simulink model "gmp_pmsm_sil_mdl"  (R2024b)
settings: Solver=VariableStepAuto  StartTime=0.0  StopTime=2  RelTol=1e-3
libraries: peripheral_utilities x11, spsSeriesRLCBranchLib x6, spsControlledVoltageSourceLib x1, gmp_sil_core_pack x1, spsGroundLib x1, spsPermanentMagnetSynchronousMachineLib x1, sps_lib x1, spspowerguiLib x1
settings Model: Creator=javnson  LastModifiedBy=javnson
settings OptimizationCC: ReuseModelBlockBuffer=off
settings RTWCC: GPUComputeCapability=3.5

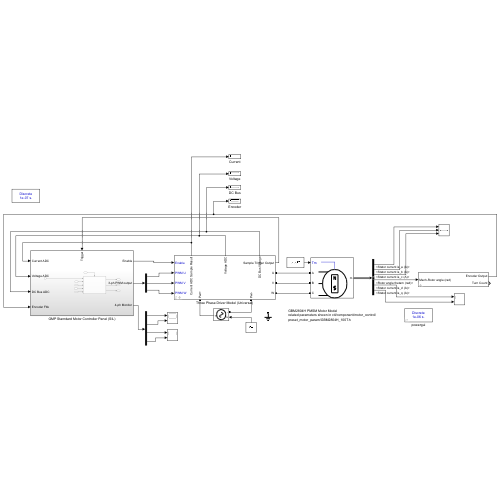
[thumbnail: Simulink's stored preview of the top-level diagram]
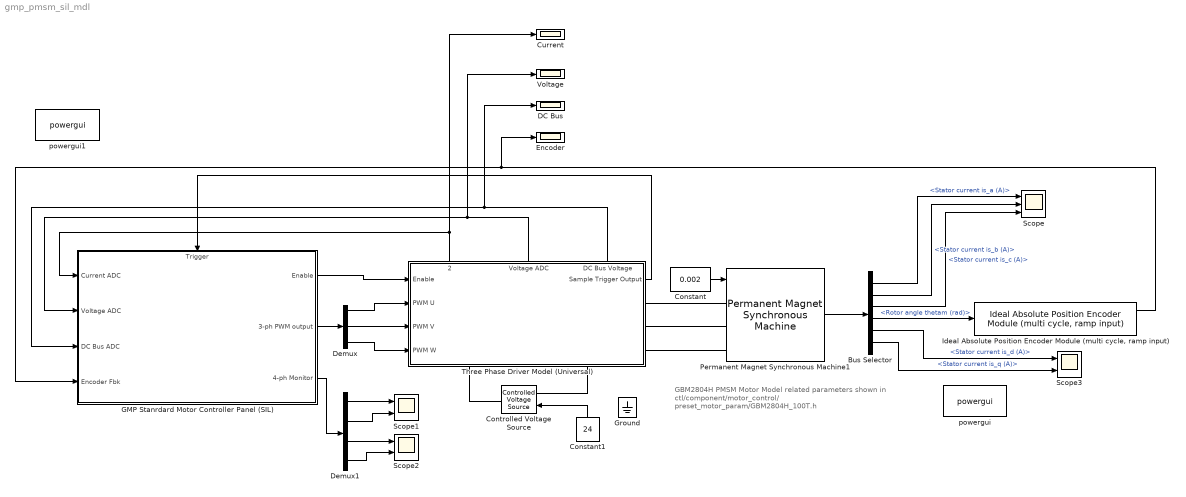
== system gmp_pmsm_sil_mdl ==
  note: GBM2804H PMSM Motor Model
      | related parameters shown in ctl/component/motor_control/
      | preset_motor_param/GBM2804H_100T.h
  Bus Selector : BusSelector  OutputSignals=Stator current is_a (A),Stator current is_b (A),Stator current is_c (A),Rotor angle thetam (rad),Stator current is_d (A),Stator current is_q (A)
  Constant : Constant  Value=0.002
  Constant1 : Constant  Value=24
  Controlled Voltage Source : spsControlledVoltageSourceLib/Controlled Voltage Source  Initialize=on  Source_Type=AC  Amplitude=0  Phase=0  Frequency=0  Measurements=None
  Current : Scope
  DC Bus : Scope
  Demux : Demux  Outputs=3
  Demux1 : Demux
  Encoder : Scope
  GMP Stanrdard Motor Controller Panel (SIL) : Subsystem
      settings: PortSchema="{\"entries\":[{\"content\":{\"sides\":[{\"content\":{\"connectorIds\":[\"In1\",\"In2\",\"In3\",\"In4\"]},\"type\":\"ConnectorPlacement.EquallySpacedRectSide\",\"uuid\":\"92070e77-c4d8-4bd6-a20f-015d90d53703\"},{\"content\":{\"connectorIds\":[\"Out1\",\"Out2\",\"Out3\"],\"side\":\"RIGHT\"},\"type\":\"ConnectorPlacement.EquallySpacedRectSide\",\"uuid\":\"cd227558-01ea-4976-b12d-cc815f5c8239\"},{\"content\":{\"connectorIds\":[\"In5\"],\"side\":\"TOP\"},\"type\":\"ConnectorPlacement.EquallySpacedRectSide\",\"uuid\":\"6d86fdab-8964-4d81-bb99-d1a603f01c68\"}]},\"type\":\"ConnectorPlacement.EquallySpacedConnector\",\"uuid\":\"4dd76185-b108-46e1-8d6d-0c6e9edd0ad4\"}],\"packageUris\":[\"http://schema.mathworks.com/mf0/Connector/R2020b\"],\"version\":\"1.0\"}"
  Ground : spsGroundLib/Ground  LConnTagsString=a
  "Ideal Absolute Position Encoder Module (multi cycle, ramp input)" : peripheral_utilities/Ideal Absolute Position Encoder Module (multi cycle, ramp input)  ENCODER_BIT=14
      settings: SourceProductName=Virtual Peripheral Utilities
  Permanent Magnet Synchronous Machine1 : spsPermanentMagnetSynchronousMachineLib/Permanent Magnet Synchronous Machine  NbPhases=3  FluxDistribution=Sinusoidal  RotorType=Round  MechanicalLoad=Torque Tm  PresetModel=No  ShowDetailedParameters=on  MeasurementBus=off  Resistance=4.7  Inductance=8.5e-3  dqInductances=[8.5e-3,8.5e-3]  La=0.96e-3  MachineConstant=Voltage Constant (V_peak L-L / krpm)  Flux=0.0038197  VoltageCst=1000/206.2  TorqueCst=0.040106  Flat=120  Mechanical=[497e-9 755e-9 7 0]  PolePairs=4  InitialConditions=[0, 0, 0, 0]  InitialConditions5ph=[0 0 0 0 0 0]  RefAngle=Aligned with phase A axis (original Park)  IterativeDiscreteModel=Trapezoidal non iterative  TsBlock=-1  TsPowergui=0
  Scope : Scope  NumInputPorts=3
  Scope1 : Scope  NumInputPorts=2
  Scope2 : Scope  NumInputPorts=2
  Scope3 : Scope  NumInputPorts=2
  Three Phase Driver Model (Universal) : Subsystem  AncestorBlock=peripheral_utilities/Three Phase Driver Model (Universal)  mask{fswitch=10e3, CMP_MAX=6000, Deadband_Upper=75, Deadband_Lower=75, Deadband_us=1.25, phase_shift=0, R_mosfet_on=0.1, Lon=0, Rd=0.01, Vf=0.3, Rs=1e5, Cs=inf, Rsap=0.005, ADC_GAIN=20, ADC_BIT=12, ADC_REFERENCE=3.3, ADC_BIAS=1.65, ADC_INIT=0, VOLTAGE_ADC_GAIN=0.04049127, VOLTAGE_ADC_BIT=12, VOLTAGE_ADC_REFERENCE=3.3, VOLTAGE_ADC_VOLTAGE=0, VOLTAGE_ADC_INIT=0, VOLTAGE_ADC_CUT_FREQ=1143.4, DCBUS_ADC_GAIN=0.04049127, DCBUS_ADC_BIT=12, DCBUS_ADC_REFERENCE=3.3, DCBUS_ADC_BIAS=0, DCBUS_ADC_INIT=0}
      mask init:
      | calculate_deadband(gcb, 'Deadband_Upper', 'Deadband_Lower',	'CMP_MAX', 'fswitch', 'Deadband_us');
      settings: PortSchema="{\"entries\":[{\"content\":{\"sides\":[{\"content\":{\"connectorIds\":[\"In1\",\"In2\",\"In3\",\"In4\"]},\"type\":\"ConnectorPlacement.EquallySpacedRectSide\",\"uuid\":\"3f4c86ad-0582-4f47-8583-a8af9a7f9adc\"},{\"content\":{\"connectorIds\":[\"Out1\",\"RConn1\",\"RConn2\",\"RConn3\"],\"side\":\"RIGHT\"},\"type\":\"ConnectorPlacement.EquallySpacedRectSide\",\"uuid\":\"ae91f325-3014-4188-9063-296f4d5623fa\"},{\"content\":{\"connectorIds\":[\"Out2\",\"Out3\",\"Out4\"],\"side\":\"TOP\"},\"type\":\"ConnectorPlacement.EquallySpacedRectSide\",\"uuid\":\"5f2edb36-6849-4a72-b7bd-4d267f120ce4\"},{\"content\":{\"connectorIds\":[\"RConn4\",\"RConn5\"],\"side\":\"BOTTOM\"},\"type\":\"ConnectorPlacement.EquallySpacedRectSide\",\"uuid\":\"79a111ed-6591-4ced-9242-67ea1247c580\"}]},\"type\":\"ConnectorPlacement.EquallySpacedConnector\",\"uuid\":\"8c66eb8e-d25c-472f-a4a5-d1759225ba1c\"}],\"packageUris\":[\"http://schema.mathworks.com/mf0/Connector/R2020b\"],\"version\":\"1.0\"}"
      mask Callback fswitch: calculate_deadband(gcb, 'Deadband_Upper', 'Deadband_Lower',	'CMP_MAX', 'fswitch', 'Deadband_us');
      mask Callback CMP_MAX: calculate_deadband(gcb, 'Deadband_Upper', 'Deadband_Lower',	'CMP_MAX', 'fswitch', 'Deadband_us');
      mask Callback Deadband_Upper: calculate_deadband(gcb, 'Deadband_Upper', 'Deadband_Lower',	'CMP_MAX', 'fswitch', 'Deadband_us');
      mask Callback Deadband_Lower: calculate_deadband(gcb, 'Deadband_Upper', 'Deadband_Lower',	'CMP_MAX', 'fswitch', 'Deadband_us');
      mask DialogControl DescGroupVar Prompt: Three Phases Bridge Peripheral(3-shunt sample)
      mask DialogControl Control21 Prompt: GMP CTL Simulink Utilities: virtual peripherals
      mask DialogControl DescTextVar Prompt: This module provide a ideal 3-phases bridge peripheral.
      mask DialogControl Container4 Prompt: PWM config
      mask DialogControl ParameterGroupVar Prompt: PWM parameters
      mask DialogControl Control2 Prompt: PWM Frequency (Hz):
      mask DialogControl Control4 Prompt: Full Scale PWM Compare value:
      mask DialogControl Control5 Prompt: Deadband Range Set (CMP Value):
      mask DialogControl Control6 Prompt: Deadband time: DEADBAND_CMP/2/CMP_MAX/fswitch
      mask DialogControl Control22 Prompt: Calculated Deadband, us
      mask DialogControl Control20 Prompt: Initial Phase shift:
      mask DialogControl Container5 Prompt: MOSFET config
      mask DialogControl Container7 Prompt: MOSFET parameters
      mask DialogControl Control7 Prompt: Rds(on), unit Ohm
      mask DialogControl Control8 Prompt: Internal diode inducctance, unit H
      mask DialogControl Control9 Prompt: Internal diode resistance Rd, unit Ohm
      mask DialogControl Control10 Prompt: Internal diode forward voltage Vf, unit V
      mask DialogControl Control11 Prompt: Snubber resistance Rs, unit ohm
      mask DialogControl Control12 Prompt: Snubber Capacitance Cs, unit F
      mask DialogControl Container6 Prompt: 3-shunt Current Sample
      mask DialogControl Control13 Prompt: ADC(p.u.) = (real_voltage * ADC_GAIN + ADC_BIAS)/ADC_REFERENCE
      mask DialogControl Control15 Prompt: Shunt Smaple Res, unit Ohm
      mask DialogControl Control14 Prompt: ADC Voltage Gain (Scale Factor):
      mask DialogControl Control16 Prompt: ADC resolution:
      mask DialogControl Control17 Prompt: ADC reference Voltage(V)
      mask DialogControl Control18 Prompt: ADC Bias Voltage(V)
      mask DialogControl Control19 Prompt: ADC Initial Voltage Output (V):
      mask DialogControl Container9 Prompt: 3-shunt Voltage Sample
      mask DialogControl Control34 Prompt: ADC Voltage Gain (Scale Factor):
      mask DialogControl Control23 Prompt: ADC resolution:
      mask DialogControl Control24 Prompt: ADC reference voltage (V), when VOLTAGE_ADC_GAIN = 1, ADC_REF = ADC Full scale
      mask DialogControl Control25 Prompt: ADC Bias Voltage (V):
      mask DialogControl Control26 Prompt: ADC Initial Voltage Output (V):
      mask DialogControl Control27 Prompt: Voltage Filter cut frequency (Hz):
      mask DialogControl Control28 Prompt: Generally, this value less than switch frequency / 10, greater than motor normal frequency * 3
      mask DialogControl Container10 Prompt: DC Bus Voltage Sample
      mask DialogControl Control32 Prompt: ADC reference voltage (V), when VOLTAGE_ADC_GAIN = 1, ADC_REF = ADC Full scale
      mask DialogControl Control29 Prompt: ADC Voltage Gain (Scale Factor):
      mask DialogControl Control30 Prompt: ADC resolution:
      mask DialogControl Control31 Prompt: ADC Bias Voltage (V):
      mask DialogControl Control33 Prompt: ADC Initial Voltage Output (V):
  Voltage : Scope
  powergui : sps_lib/powergui  Priority=1  SimulationMode=Discrete  SampleTime=1e-6  frequency=60  Iterations=50  frequencyindice=0  Pbase=100e6  ErrMax=1e-4  UnitsV=kV  UnitsW=MW  buscounter=0  FunctionMessages=off  echomessages=off  EnableUseOfTLC=off  CurrentSourceSwitches=off  DisableSnubberDevices=off  DisableRonSwitches=off  DisableVfSwitches=off  DisplayEquations=off  AutomaticDiscreteSolvers=off  SolverType=Tustin/Backward Euler (TBE)  Interpol=off  ExternalGateDelay=off  methode=off  Ts=100  x0status=blocks  SPID=on  SwTol=0  HookPort=off  NonlinearTolerance=1e-4  nMaxIteration=100  ContinueOnMaxIteration=off  RestoreLinks=warning  ResistiveCurrentMeasurement=off  Frange=[0:2:500]  Ylog=off  Xlog=on  ShowGrid=off  save=off  variable=ZData  structure=0  ZoomFFT=off  StartTime=0.0  cycles=1  DisplayStyle=1  fundamental=60  FreqAxis=off  MaxFrequency=1000  frequencyindicesteady=1  RmsSteady=1  display=off
  powergui1 : spspowerguiLib/powergui  Priority=1  SimulationMode=Discrete  SampleTime=1e-7  frequency=60  Iterations=50  frequencyindice=60  Pbase=100e6  ErrMax=1e-4  UnitsV=kV  UnitsW=MW  buscounter=0  FunctionMessages=off  echomessages=off  EnableUseOfTLC=off  CurrentSourceSwitches=off  DisableSnubberDevices=off  DisableRonSwitches=off  DisableVfSwitches=off  DisplayEquations=off  AutomaticDiscreteSolvers=off  SolverType=Tustin/Backward Euler (TBE)  Interpol=off  ExternalGateDelay=off  methode=off  Ts=100  x0status=blocks  SPID=on  SwTol=0  HookPort=off  NonlinearTolerance=1e-4  nMaxIteration=100  ContinueOnMaxIteration=off  RestoreLinks=warning  ResistiveCurrentMeasurement=off  Frange=[0:2:500]  Ylog=off  Xlog=on  ShowGrid=off  save=off  variable=ZData  structure=0  ZoomFFT=off  StartTime=0.0  cycles=1  DisplayStyle=1  fundamental=60  FreqAxis=off  MaxFrequency=1000  frequencyindicesteady=1  RmsSteady=1  display=off
  wires:
  Constant/1 -> Permanent Magnet Synchronous Machine1/1
  Bus Selector/1 -> Scope/1  "<Stator current is_a (A)>"
  Bus Selector/2 -> Scope/2  "<Stator current is_b (A)>"
  Bus Selector/3 -> Scope/3  "<Stator current is_c (A)>"
  Demux/1 -> Three Phase Driver Model (Universal)/2(PWM U)
  Demux/2 -> Three Phase Driver Model (Universal)/3(PWM V)
  Demux/3 -> Three Phase Driver Model (Universal)/4(PWM W)
  Constant1/1 -> Controlled Voltage Source/1
  Bus Selector/4 -> "Ideal Absolute Position Encoder Module (multi cycle, ramp input)"/1  "<Rotor angle thetam (rad)>"
  Three Phase Driver Model (Universal)/2(Current ADC Sample Result) -> Current/1, GMP Stanrdard Motor Controller Panel (SIL)/1(Current ADC)
  Three Phase Driver Model (Universal)/3(Voltage ADC) -> Voltage/1, GMP Stanrdard Motor Controller Panel (SIL)/2(Voltage ADC)
  "Ideal Absolute Position Encoder Module (multi cycle, ramp input)"/1 -> GMP Stanrdard Motor Controller Panel (SIL)/4(Encoder Fbk), Encoder/1
  GMP Stanrdard Motor Controller Panel (SIL)/1(Enable) -> Three Phase Driver Model (Universal)/1(Enable)
  GMP Stanrdard Motor Controller Panel (SIL)/2(3-ph PWM output) -> Demux/1
  GMP Stanrdard Motor Controller Panel (SIL)/3(4-ph Monitor) -> Demux1/1
  Three Phase Driver Model (Universal)/1(Sample Trigger Output) -> GMP Stanrdard Motor Controller Panel (SIL)/5(Trigger)
  Three Phase Driver Model (Universal)/4(DC Bus Voltage) -> GMP Stanrdard Motor Controller Panel (SIL)/3(DC Bus ADC), DC Bus/1
  Permanent Magnet Synchronous Machine1/1 -> Bus Selector/1
  Demux1/1 -> Scope1/1
  Demux1/2 -> Scope1/2
  Demux1/3 -> Scope2/1
  Demux1/4 -> Scope2/2
  Bus Selector/5 -> Scope3/1  "<Stator current is_d (A)>"
  Bus Selector/6 -> Scope3/2  "<Stator current is_q (A)>"
  connections:
  Permanent Magnet Synchronous Machine1/LConn1 -- Three Phase Driver Model (Universal)/RConn1
  Permanent Magnet Synchronous Machine1/LConn2 -- Three Phase Driver Model (Universal)/RConn2
  Permanent Magnet Synchronous Machine1/LConn3 -- Three Phase Driver Model (Universal)/RConn3
  Three Phase Driver Model (Universal)/RConn4 -- Controlled Voltage Source/RConn1
  Three Phase Driver Model (Universal)/RConn5 -- Controlled Voltage Source/LConn1

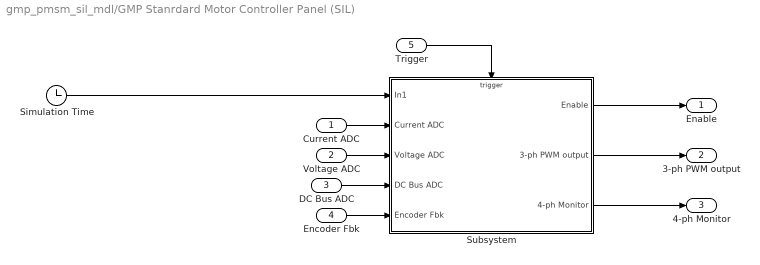
== system gmp_pmsm_sil_mdl/GMP Stanrdard Motor Controller Panel (SIL) ==
  Current ADC : Inport
  Voltage ADC : Inport  Port=2
  DC Bus ADC : Inport  Port=3
  Encoder Fbk : Inport  Port=4
  Trigger : Inport  Port=5
  Simulation Time : Clock
  Subsystem : Subsystem
  Enable : Outport
  3-ph PWM output : Outport  Port=2
  4-ph Monitor : Outport  Port=3
  wires:
  Simulation Time/1 -> Subsystem/1(In1)
  Current ADC/1 -> Subsystem/2(Current ADC)
  Voltage ADC/1 -> Subsystem/3(Voltage ADC)
  DC Bus ADC/1 -> Subsystem/4(DC Bus ADC)
  Encoder Fbk/1 -> Subsystem/5(Encoder Fbk)
  Subsystem/1(Enable) -> Enable/1
  Subsystem/2(3-ph PWM output) -> 3-ph PWM output/1
  Subsystem/3(4-ph Monitor) -> 4-ph Monitor/1
  Trigger/1 -> Subsystem/Trigger

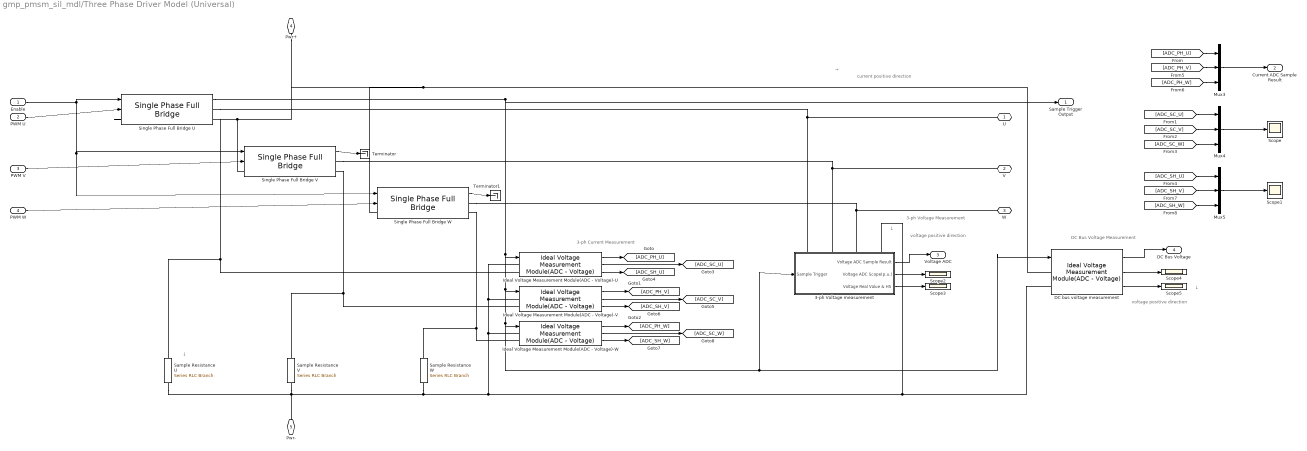
== system gmp_pmsm_sil_mdl/Three Phase Driver Model (Universal) ==
  note: voltage positive direction
  note: ↓
  note: DC Bus Voltage Measurement
  note: 3-ph Voltage Measurement
  note: ↓
  note: voltage positive direction
  note: ↓
  note: current positive direction
  note: →
  note: 3-ph Current Measurement
  Enable : Inport
  PWM U : Inport  Port=2
  PWM V : Inport  Port=3
  PWM W : Inport  Port=4
  3-ph Voltage measurement : Subsystem  AncestorBlock=peripheral_utilities/Three Phases Voltage (ph-gnd) Measurement with Filter  mask{ADC_GAIN=VOLTAGE_ADC_GAIN, ADC_BIT=VOLTAGE_ADC_BIT, ADC_REFERENCE=VOLTAGE_ADC_REFERENCE, ADC_BIAS=VOLTAGE_ADC_VOLTAGE, ADC_INIT=VOLTAGE_ADC_INIT, cut_frequency=VOLTAGE_ADC_CUT_FREQ}
      settings: PortSchema="{\"entries\":[{\"content\":{\"sides\":[{\"content\":{\"connectorIds\":[\"In1\"]},\"type\":\"ConnectorPlacement.EquallySpacedRectSide\",\"uuid\":\"ae4f4612-c092-4fa0-8a43-5c9e823110e3\"},{\"content\":{\"connectorIds\":[\"Out1\",\"Out2\",\"Out3\"],\"side\":\"RIGHT\"},\"type\":\"ConnectorPlacement.EquallySpacedRectSide\",\"uuid\":\"6db15ef0-d33a-4775-b4e6-14a566796673\"},{\"content\":{\"connectorIds\":[\"LConn1\",\"LConn2\",\"LConn3\",\"LConn4\"],\"side\":\"TOP\"},\"type\":\"ConnectorPlacement.EquallySpacedRectSide\",\"uuid\":\"cfddd664-59f3-497b-b33e-fe832fe7a7bd\"}]},\"type\":\"ConnectorPlacement.EquallySpacedConnector\",\"uuid\":\"5bacf0ad-0c4a-4f47-a242-d8a476ab7f52\"}],\"packageUris\":[\"http://schema.mathworks.com/mf0/Connector/R2020b\"],\"version\":\"1.0\"}"
      mask DialogControl DescGroupVar Prompt: 3 phases Voltage Sample ADC Model
      mask DialogControl Control10 Prompt: GMP CTL Simulink Utilities: virtual peripherals
      mask DialogControl DescTextVar Prompt: This is a ideal Voltage Measurement Module.
      mask DialogControl Control2 Prompt: ADC(p.u.) = (real_voltage * ADC_GAIN + ADC_BIAS)/ADC_REFERENCE
      mask DialogControl ParameterGroupVar Prompt: parameters:
      mask DialogControl Control3 Prompt: ADC Voltage Gain (Scale Factor):
      mask DialogControl Control4 Prompt: ADC resolution:
      mask DialogControl Control5 Prompt: ADC reference Voltage (V), when ADC_GAIN=1, ADC_REF = ADC full scale
      mask DialogControl Control6 Prompt: ADC Bias Voltage(V)
      mask DialogControl Control7 Prompt: ADC Initial Voltage Output (V):
      mask DialogControl Control8 Prompt: Voltage Filter cut frequency (Hz):
      mask DialogControl Control9 Prompt: Generally, this value less than switch frequency / 10, greater than motor normal frequency * 3
  DC bus voltage measurement : peripheral_utilities/Ideal Voltage Measurement Module(ADC - Voltage)  ADC_GAIN=DCBUS_ADC_GAIN  ADC_BIT=DCBUS_ADC_BIT  ADC_REFERENCE=DCBUS_ADC_REFERENCE  ADC_BIAS=DCBUS_ADC_BIAS  ADC_INIT=DCBUS_ADC_INIT
      settings: SourceProductName=Virtual Peripheral Utilities
  Ideal Voltage Measurement Module(ADC - Voltage)-U : peripheral_utilities/Ideal Voltage Measurement Module(ADC - Voltage)  ADC_GAIN=ADC_GAIN  ADC_BIT=ADC_BIT  ADC_REFERENCE=ADC_REFERENCE  ADC_BIAS=ADC_BIAS  ADC_INIT=ADC_INIT
      settings: SourceProductName=Virtual Peripheral Utilities
  Ideal Voltage Measurement Module(ADC - Voltage)-V : peripheral_utilities/Ideal Voltage Measurement Module(ADC - Voltage)  ADC_GAIN=ADC_GAIN  ADC_BIT=ADC_BIT  ADC_REFERENCE=ADC_REFERENCE  ADC_BIAS=ADC_BIAS  ADC_INIT=ADC_INIT
      settings: SourceProductName=Virtual Peripheral Utilities
  Ideal Voltage Measurement Module(ADC - Voltage)-W : peripheral_utilities/Ideal Voltage Measurement Module(ADC - Voltage)  ADC_GAIN=ADC_GAIN  ADC_BIT=ADC_BIT  ADC_REFERENCE=ADC_REFERENCE  ADC_BIAS=ADC_BIAS  ADC_INIT=ADC_INIT
      settings: SourceProductName=Virtual Peripheral Utilities
  Mux3 : Mux  Inputs=3
  Mux4 : Mux  Inputs=3
  Mux5 : Mux  Inputs=3
  Sample Resistance U : spsSeriesRLCBranchLib/Series RLC Branch  LConnTagsString=__new0  RConnTagsString=__new0  BranchType=R  Resistance=Rsap  Inductance=1e-3  SetiL0=off  InitialCurrent=0  Capacitance=1e-6  Setx0=off  InitialVoltage=0  Measurements=None
  Sample Resistance V : spsSeriesRLCBranchLib/Series RLC Branch  LConnTagsString=__new0  RConnTagsString=__new0  BranchType=R  Resistance=Rsap  Inductance=1e-3  SetiL0=off  InitialCurrent=0  Capacitance=1e-6  Setx0=off  InitialVoltage=0  Measurements=None
  Sample Resistance W : spsSeriesRLCBranchLib/Series RLC Branch  LConnTagsString=__new0  RConnTagsString=__new0  BranchType=R  Resistance=Rsap  Inductance=1e-3  SetiL0=off  InitialCurrent=0  Capacitance=1e-6  Setx0=off  InitialVoltage=0  Measurements=None
  Scope{,1..5} (6 alike) : Scope
  Single Phase Full Bridge U : peripheral_utilities/Single Phase Full Bridge  fswitch=fswitch  CMP_MAX=CMP_MAX  Deadband_Upper=Deadband_Upper  Deadband_Lower=Deadband_Lower  Deadband_us=NaN  phase_shift=phase_shift  R_mosfet_on=R_mosfet_on  Lon=Lon  Rd=Rd  Vf=Vf  Rs=Rs  Cs=Cs
      settings: SourceProductName=Virtual Peripheral Utilities
  Single Phase Full Bridge V : peripheral_utilities/Single Phase Full Bridge  fswitch=fswitch  CMP_MAX=CMP_MAX  Deadband_Upper=Deadband_Upper  Deadband_Lower=Deadband_Lower  Deadband_us=NaN  phase_shift=phase_shift  R_mosfet_on=R_mosfet_on  Lon=Lon  Rd=Rd  Vf=Vf  Rs=Rs  Cs=Cs
      settings: SourceProductName=Virtual Peripheral Utilities
  Single Phase Full Bridge W : peripheral_utilities/Single Phase Full Bridge  fswitch=fswitch  CMP_MAX=CMP_MAX  Deadband_Upper=Deadband_Upper  Deadband_Lower=Deadband_Lower  Deadband_us=NaN  phase_shift=phase_shift  R_mosfet_on=R_mosfet_on  Lon=Lon  Rd=Rd  Vf=Vf  Rs=Rs  Cs=Cs
      settings: SourceProductName=Virtual Peripheral Utilities
  Terminator : Terminator
  Terminator1 : Terminator
  U : PMIOPort  Side=Right
  V : PMIOPort  Port=2  Side=Right
  W : PMIOPort  Port=3  Side=Right
  Pwr+ : PMIOPort  Port=4  Side=Right
  Pwr- : PMIOPort  Port=5  Side=Right
  Sample Trigger Output : Outport
  Current ADC Sample Result : Outport  Port=2
  Voltage ADC : Outport  Port=3
  DC Bus Voltage : Outport  Port=4
  wires:
  DC bus voltage measurement/3 -> Scope5/1
  DC bus voltage measurement/2 -> Scope4/1
  DC bus voltage measurement/1 -> DC Bus Voltage/1
  3-ph Voltage measurement/3(Voltage Real Value & HS) -> Scope3/1
  3-ph Voltage measurement/2(Voltage ADC Scope(p.u.)) -> Scope2/1
  3-ph Voltage measurement/1(Voltage ADC Sample Result) -> Voltage ADC/1
  Ideal Voltage Measurement Module(ADC - Voltage)-W/2 -> [ADC_SC_W]
  [ADC_SH_V] -> Mux5/2
  [ADC_SC_W] -> Mux4/3
  [ADC_PH_W] -> Mux3/3
  Ideal Voltage Measurement Module(ADC - Voltage)-W/3 -> [ADC_SH_W]
  Ideal Voltage Measurement Module(ADC - Voltage)-V/2 -> [ADC_SC_V]
  [ADC_SH_U] -> Mux5/1
  Single Phase Full Bridge U/1 -> Sample Trigger Output/1, Ideal Voltage Measurement Module(ADC - Voltage)-U/1, 3-ph Voltage measurement/1(Sample Trigger), DC bus voltage measurement/1, Ideal Voltage Measurement Module(ADC - Voltage)-W/1, Ideal Voltage Measurement Module(ADC - Voltage)-V/1
  Ideal Voltage Measurement Module(ADC - Voltage)-V/3 -> [ADC_SH_V]
  Mux4/1 -> Scope/1
  Enable/1 -> Single Phase Full Bridge U/1, Single Phase Full Bridge W/1, Single Phase Full Bridge V/1
  [ADC_PH_U] -> Mux3/1
  Ideal Voltage Measurement Module(ADC - Voltage)-W/1 -> [ADC_PH_W]
  Mux5/1 -> Scope1/1
  [ADC_SH_W] -> Mux5/3
  [ADC_SC_U] -> Mux4/1
  Ideal Voltage Measurement Module(ADC - Voltage)-V/1 -> [ADC_PH_V]
  Mux3/1 -> Current ADC Sample Result/1
  Ideal Voltage Measurement Module(ADC - Voltage)-U/3 -> [ADC_SH_U]
  [ADC_SC_V] -> Mux4/2
  [ADC_PH_V] -> Mux3/2
  PWM W/1 -> Single Phase Full Bridge W/2
  PWM V/1 -> Single Phase Full Bridge V/2
  Ideal Voltage Measurement Module(ADC - Voltage)-U/2 -> [ADC_SC_U]
  Single Phase Full Bridge W/1 -> Terminator1/1
  Single Phase Full Bridge V/1 -> Terminator/1
  Ideal Voltage Measurement Module(ADC - Voltage)-U/1 -> [ADC_PH_U]
  PWM U/1 -> Single Phase Full Bridge U/2
  connections:
  Single Phase Full Bridge V/LConn1 -- Single Phase Full Bridge U/LConn1 -- DC bus voltage measurement/LConn1 -- Single Phase Full Bridge W/LConn1 -- Pwr+/RConn1
  Single Phase Full Bridge U/RConn2 -- Ideal Voltage Measurement Module(ADC - Voltage)-U/LConn2 -- Sample Resistance U/LConn1
  Single Phase Full Bridge W/RConn2 -- Ideal Voltage Measurement Module(ADC - Voltage)-W/LConn2 -- Sample Resistance W/LConn1
  Ideal Voltage Measurement Module(ADC - Voltage)-W/LConn1 -- Ideal Voltage Measurement Module(ADC - Voltage)-V/LConn1 -- Ideal Voltage Measurement Module(ADC - Voltage)-U/LConn1 -- DC bus voltage measurement/LConn2 -- 3-ph Voltage measurement/LConn4 -- Sample Resistance W/RConn1 -- Sample Resistance V/RConn1 -- Sample Resistance U/RConn1 -- Pwr-/RConn1
  Single Phase Full Bridge V/RConn2 -- Ideal Voltage Measurement Module(ADC - Voltage)-V/LConn2 -- Sample Resistance V/LConn1
  3-ph Voltage measurement/LConn3 -- W/RConn1 -- Single Phase Full Bridge W/RConn1
  3-ph Voltage measurement/LConn1 -- U/RConn1 -- Single Phase Full Bridge U/RConn1
  3-ph Voltage measurement/LConn2 -- V/RConn1 -- Single Phase Full Bridge V/RConn1

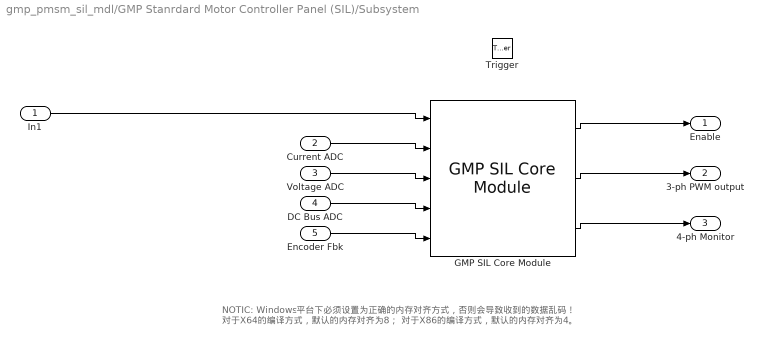
== system gmp_pmsm_sil_mdl/GMP Stanrdard Motor Controller Panel (SIL)/Subsystem ==
  note: NOTIC:
      | Windows平台下必须设置为正确的内存对齐方式，否则会导致收到的数据乱码！
      | 对于X64的编译方式，默认的内存对齐为8；
      | 对于X86的编译方式，默认的内存对齐为4。
  In1 : Inport
  Current ADC : Inport  Port=2
  Voltage ADC : Inport  Port=3
  DC Bus ADC : Inport  Port=4
  Encoder Fbk : Inport  Port=5
  Trigger : TriggerPort  VariantControl=(inherit)  PortDimensions=1
  GMP SIL Core Module : gmp_sil_core_pack/GMP SIL Core Module  MaskPackedDataTypes={'double','uint32','uint32','uint32','uint32'}  MaskPackedDataSizes={[1],[3],[3],[1],[1]}  MaskUnpackedDataTypes={'double', 'uint32','double'}  MaskUnpackedDataSizes={[1],[3],[4]}  MaskAlignment=1  MaskHostAddr='127.0.0.1'  MaskMsgTxPort=12300  MaskMsgRxPort=12301  MaskCmdTxPort=12302  MaskCmdRxPort=12303
      settings: SourceProductName=GMP SIL Core Utilities
  Enable : Outport
  3-ph PWM output : Outport  Port=2
  4-ph Monitor : Outport  Port=3
  wires:
  Encoder Fbk/1 -> GMP SIL Core Module/5
  Current ADC/1 -> GMP SIL Core Module/2
  Voltage ADC/1 -> GMP SIL Core Module/3
  DC Bus ADC/1 -> GMP SIL Core Module/4
  In1/1 -> GMP SIL Core Module/1
  GMP SIL Core Module/3 -> 4-ph Monitor/1
  GMP SIL Core Module/2 -> 3-ph PWM output/1
  GMP SIL Core Module/1 -> Enable/1

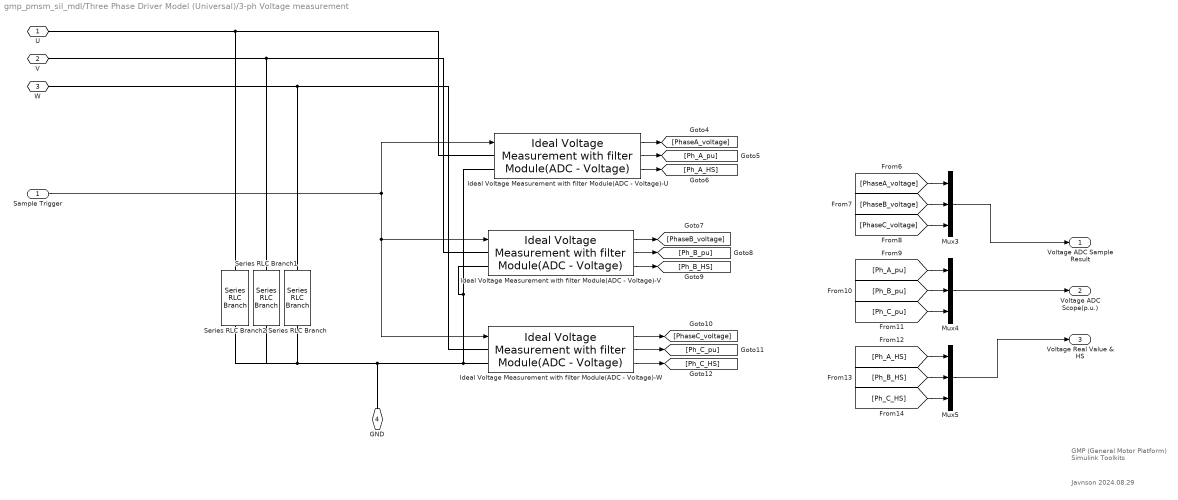
== system gmp_pmsm_sil_mdl/Three Phase Driver Model (Universal)/3-ph Voltage measurement ==
  note: GMP (General Motor Platform)
      | Simulink Toolkits
  note: Javnson
      | 2024.08.29
  Sample Trigger : Inport
  Ideal Voltage Measurement with filter Module(ADC - Voltage)-U : peripheral_utilities/Ideal Voltage Measurement with filter Module(ADC - Voltage)  ADC_GAIN=ADC_GAIN  ADC_BIT=ADC_BIT  ADC_REFERENCE=ADC_REFERENCE  ADC_BIAS=ADC_BIAS  ADC_INIT=ADC_INIT  cut_frequency=cut_frequency
      settings: SourceProductName=Virtual Peripheral Utilities
  Ideal Voltage Measurement with filter Module(ADC - Voltage)-V : peripheral_utilities/Ideal Voltage Measurement with filter Module(ADC - Voltage)  ADC_GAIN=ADC_GAIN  ADC_BIT=ADC_BIT  ADC_REFERENCE=ADC_REFERENCE  ADC_BIAS=ADC_BIAS  ADC_INIT=ADC_INIT  cut_frequency=cut_frequency
      settings: SourceProductName=Virtual Peripheral Utilities
  Ideal Voltage Measurement with filter Module(ADC - Voltage)-W : peripheral_utilities/Ideal Voltage Measurement with filter Module(ADC - Voltage)  ADC_GAIN=ADC_GAIN  ADC_BIT=ADC_BIT  ADC_REFERENCE=ADC_REFERENCE  ADC_BIAS=ADC_BIAS  ADC_INIT=ADC_INIT  cut_frequency=cut_frequency
      settings: SourceProductName=Virtual Peripheral Utilities
  Mux3 : Mux  Inputs=3
  Mux4 : Mux  Inputs=3
  Mux5 : Mux  Inputs=3
  Series RLC Branch : spsSeriesRLCBranchLib/Series RLC Branch  LConnTagsString=__new0  RConnTagsString=__new0  BranchType=R  Resistance=1e6  Inductance=1e-3  SetiL0=off  InitialCurrent=0  Capacitance=1e-6  Setx0=off  InitialVoltage=0  Measurements=None
  Series RLC Branch1 : spsSeriesRLCBranchLib/Series RLC Branch  LConnTagsString=__new0  RConnTagsString=__new0  BranchType=R  Resistance=1e6  Inductance=1e-3  SetiL0=off  InitialCurrent=0  Capacitance=1e-6  Setx0=off  InitialVoltage=0  Measurements=None
  Series RLC Branch2 : spsSeriesRLCBranchLib/Series RLC Branch  LConnTagsString=__new0  RConnTagsString=__new0  BranchType=R  Resistance=1e6  Inductance=1e-3  SetiL0=off  InitialCurrent=0  Capacitance=1e-6  Setx0=off  InitialVoltage=0  Measurements=None
  U : PMIOPort  Side=Left
  V : PMIOPort  Port=2  Side=Left
  W : PMIOPort  Port=3  Side=Left
  GND : PMIOPort  Port=4  Side=Left
  Voltage ADC Sample Result : Outport
  Voltage ADC Scope(p.u.) : Outport  Port=2
  Voltage Real Value & HS : Outport  Port=3
  wires:
  Mux5/1 -> Voltage Real Value & HS/1
  [Ph_A_HS] -> Mux5/1
  Mux3/1 -> Voltage ADC Sample Result/1
  [Ph_C_HS] -> Mux5/3
  [Ph_C_pu] -> Mux4/3
  [PhaseA_voltage] -> Mux3/1
  [PhaseC_voltage] -> Mux3/3
  [Ph_A_pu] -> Mux4/1
  Ideal Voltage Measurement with filter Module(ADC - Voltage)-W/2 -> [Ph_C_pu]
  Ideal Voltage Measurement with filter Module(ADC - Voltage)-U/3 -> [Ph_A_HS]
  [PhaseB_voltage] -> Mux3/2
  [Ph_B_pu] -> Mux4/2
  Ideal Voltage Measurement with filter Module(ADC - Voltage)-U/2 -> [Ph_A_pu]
  Ideal Voltage Measurement with filter Module(ADC - Voltage)-U/1 -> [PhaseA_voltage]
  Ideal Voltage Measurement with filter Module(ADC - Voltage)-V/1 -> [PhaseB_voltage]
  Ideal Voltage Measurement with filter Module(ADC - Voltage)-W/1 -> [PhaseC_voltage]
  [Ph_B_HS] -> Mux5/2
  Mux4/1 -> Voltage ADC Scope(p.u.)/1
  Ideal Voltage Measurement with filter Module(ADC - Voltage)-V/3 -> [Ph_B_HS]
  Ideal Voltage Measurement with filter Module(ADC - Voltage)-V/2 -> [Ph_B_pu]
  Sample Trigger/1 -> Ideal Voltage Measurement with filter Module(ADC - Voltage)-V/1, Ideal Voltage Measurement with filter Module(ADC - Voltage)-W/1, Ideal Voltage Measurement with filter Module(ADC - Voltage)-U/1
  Ideal Voltage Measurement with filter Module(ADC - Voltage)-W/3 -> [Ph_C_HS]
  connections:
  Ideal Voltage Measurement with filter Module(ADC - Voltage)-W/LConn1 -- Series RLC Branch/LConn1 -- W/RConn1
  Ideal Voltage Measurement with filter Module(ADC - Voltage)-V/LConn1 -- Series RLC Branch1/LConn1 -- V/RConn1
  Ideal Voltage Measurement with filter Module(ADC - Voltage)-U/LConn1 -- Series RLC Branch2/LConn1 -- U/RConn1
  Ideal Voltage Measurement with filter Module(ADC - Voltage)-W/LConn2 -- GND/RConn1 -- Series RLC Branch/RConn1 -- Series RLC Branch1/RConn1 -- Series RLC Branch2/RConn1 -- Ideal Voltage Measurement with filter Module(ADC - Voltage)-U/LConn2 -- Ideal Voltage Measurement with filter Module(ADC - Voltage)-V/LConn2
